simulink model "DCHR_Dispatch_Stateflow_v22"  (R2026a)
settings: Solver=FixedStepDiscrete  StopTime=dchr_stop_v22  FixedStep=dchr_dt_v22
model workspace (MAT data in the model file):
  dchr_E0_v22 = 0
  dchr_dt_v22 = 1
  dchr_h_v22 = [8 0.45 1.2 8 0.08 0 4 0 0]
  dchr_input_v22 = [0  6  35  70  5; 1  0  35  70  6; 2  0  35  70  10]
  dchr_p_v22 = [1 10 3 4 0.9 0.8 0.01 2]
  dchr_stop_v22 = 2
settings Model: Creator=Lysda  LastModifiedBy=Lysda

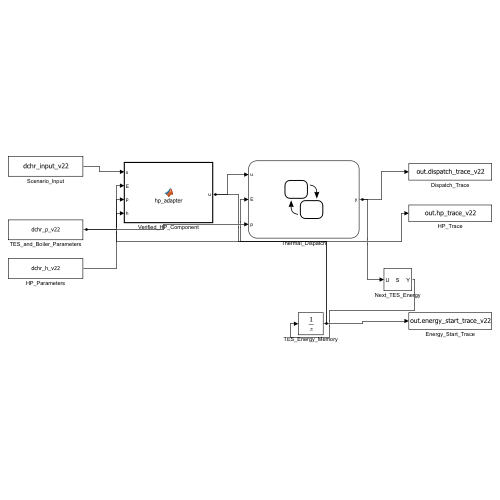
[thumbnail: Simulink's stored preview of the top-level diagram]
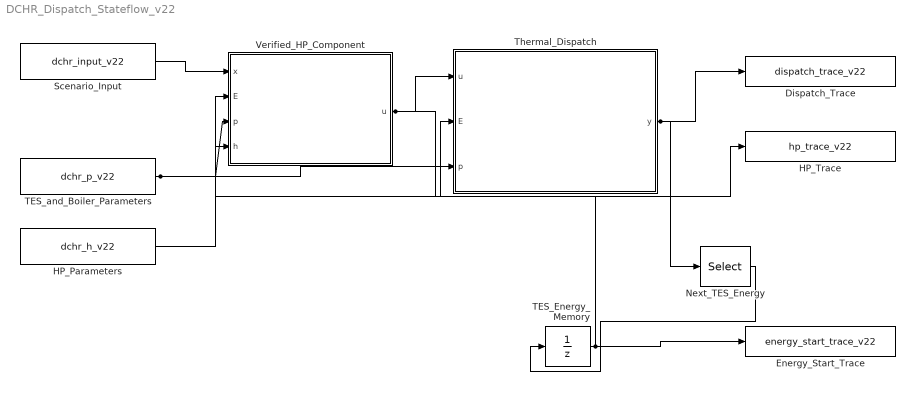
== system DCHR_Dispatch_Stateflow_v22 ==
  Dispatch_Trace : ToWorkspace  VariableName=dispatch_trace_v22  SaveFormat=Timeseries  SampleTime=-1
  Energy_Start_Trace : ToWorkspace  VariableName=energy_start_trace_v22  SaveFormat=Timeseries  SampleTime=-1
  HP_Parameters : Constant  Value=dchr_h_v22
  HP_Trace : ToWorkspace  VariableName=hp_trace_v22  SaveFormat=Timeseries  SampleTime=-1
  Next_TES_Energy : Selector  InputPortWidth=13  IndexOptions=Index vector (dialog)  Indices=8  OutputSizes=1
  Scenario_Input : FromWorkspace  VariableName=dchr_input_v22  SampleTime=dchr_dt_v22  Interpolate=off  OutputAfterFinalValue=Holding final value
  TES_Energy_Memory : UnitDelay  InitialCondition=dchr_E0_v22  SampleTime=dchr_dt_v22
  TES_and_Boiler_Parameters : Constant  Value=dchr_p_v22
  Thermal_Dispatch : Stateflow chart  TreatAsAtomicUnit=on
  Verified_HP_Component : MATLAB Function  TreatAsAtomicUnit=on
  wires:
  Scenario_Input/1 -> Verified_HP_Component/1(x)
  TES_Energy_Memory/1 -> Verified_HP_Component/2(E), Thermal_Dispatch/2(E), Energy_Start_Trace/1
  TES_and_Boiler_Parameters/1 -> Verified_HP_Component/3(p), Thermal_Dispatch/3(p)
  HP_Parameters/1 -> Verified_HP_Component/4(h)
  Verified_HP_Component/1(u) -> Thermal_Dispatch/1(u), HP_Trace/1
  Thermal_Dispatch/1(y) -> Next_TES_Energy/1, Dispatch_Trace/1
  Next_TES_Energy/1 -> TES_Energy_Memory/1

== matlab function DCHR_Dispatch_Stateflow_v22/Verified_HP_Component ==
  data: x input; u output; E input; p input; h input
function u=hp_adapter(x,E,p,h)
%#codegen
coder.extrinsic('dchr_stateflow_hp_v22');
u=zeros(8,1);
u=dchr_stateflow_hp_v22(x,E,p,h);
end

== stateflow chart DCHR_Dispatch_Stateflow_v22/Thermal_Dispatch ==
  settings: updateMethod=DISCRETE  sampleTime=dchr_dt_v22  description=v22 six-state finite TES/HP/boiler dispatch. Normal-mode host HP component; state actions drive all delivery ports.
  state IDLE
    en,du:
    y=stateflow_allocate_v22(0,u,E,p);
  state HEAT_RECOVERY
    en,du:
    y=stateflow_allocate_v22(1,u,E,p);
  state STORAGE_CHARGE
    en,du:
    y=stateflow_allocate_v22(2,u,E,p);
  state STORAGE_DISCHARGE
    en,du:
    y=stateflow_allocate_v22(3,u,E,p);
  state BACKUP
    en,du:
    y=stateflow_allocate_v22(4,u,E,p);
  state UNMET_DEMAND
    en,du:
    y=stateflow_allocate_v22(5,u,E,p);
  (junction 22) -> STORAGE_CHARGE [order 3] : [stateflow_choose_mode_v22(u,E,p)==2]
  (junction 22) -> HEAT_RECOVERY [order 2] : [stateflow_choose_mode_v22(u,E,p)==1]
  (default) -> (junction 22)
  (junction 22) -> IDLE [order 1] : [stateflow_choose_mode_v22(u,E,p)==0]
  (junction 22) -> UNMET_DEMAND [order 6] : [stateflow_choose_mode_v22(u,E,p)==5]
  (junction 22) -> STORAGE_DISCHARGE [order 4] : [stateflow_choose_mode_v22(u,E,p)==3]
  (junction 22) -> BACKUP [order 5] : [stateflow_choose_mode_v22(u,E,p)==4]
  STORAGE_CHARGE -> STORAGE_DISCHARGE [order 3] : [stateflow_choose_mode_v22(u,E,p)==3]
  HEAT_RECOVERY -> STORAGE_DISCHARGE [order 3] : [stateflow_choose_mode_v22(u,E,p)==3]
  STORAGE_CHARGE -> BACKUP [order 4] : [stateflow_choose_mode_v22(u,E,p)==4]
  STORAGE_DISCHARGE -> IDLE [order 1] : [stateflow_choose_mode_v22(u,E,p)==0]
  UNMET_DEMAND -> IDLE [order 1] : [stateflow_choose_mode_v22(u,E,p)==0]
  STORAGE_CHARGE -> IDLE [order 1] : [stateflow_choose_mode_v22(u,E,p)==0]
  BACKUP -> IDLE [order 1] : [stateflow_choose_mode_v22(u,E,p)==0]
  HEAT_RECOVERY -> IDLE [order 1] : [stateflow_choose_mode_v22(u,E,p)==0]
  STORAGE_DISCHARGE -> HEAT_RECOVERY [order 2] : [stateflow_choose_mode_v22(u,E,p)==1]
  STORAGE_DISCHARGE -> STORAGE_CHARGE [order 3] : [stateflow_choose_mode_v22(u,E,p)==2]
  BACKUP -> HEAT_RECOVERY [order 2] : [stateflow_choose_mode_v22(u,E,p)==1]
  IDLE -> HEAT_RECOVERY [order 1] : [stateflow_choose_mode_v22(u,E,p)==1]
  IDLE -> STORAGE_CHARGE [order 2] : [stateflow_choose_mode_v22(u,E,p)==2]
  UNMET_DEMAND -> HEAT_RECOVERY [order 2] : [stateflow_choose_mode_v22(u,E,p)==1]
  STORAGE_CHARGE -> HEAT_RECOVERY [order 2] : [stateflow_choose_mode_v22(u,E,p)==1]
  BACKUP -> STORAGE_CHARGE [order 3] : [stateflow_choose_mode_v22(u,E,p)==2]
  UNMET_DEMAND -> STORAGE_CHARGE [order 3] : [stateflow_choose_mode_v22(u,E,p)==2]
  HEAT_RECOVERY -> STORAGE_CHARGE [order 2] : [stateflow_choose_mode_v22(u,E,p)==2]
  IDLE -> STORAGE_DISCHARGE [order 3] : [stateflow_choose_mode_v22(u,E,p)==3]
  HEAT_RECOVERY -> BACKUP [order 4] : [stateflow_choose_mode_v22(u,E,p)==4]
  STORAGE_CHARGE -> UNMET_DEMAND [order 5] : [stateflow_choose_mode_v22(u,E,p)==5]
  IDLE -> BACKUP [order 4] : [stateflow_choose_mode_v22(u,E,p)==4]
  IDLE -> UNMET_DEMAND [order 5] : [stateflow_choose_mode_v22(u,E,p)==5]
  HEAT_RECOVERY -> UNMET_DEMAND [order 5] : [stateflow_choose_mode_v22(u,E,p)==5]
  UNMET_DEMAND -> STORAGE_DISCHARGE [order 4] : [stateflow_choose_mode_v22(u,E,p)==3]
  BACKUP -> STORAGE_DISCHARGE [order 4] : [stateflow_choose_mode_v22(u,E,p)==3]
  STORAGE_DISCHARGE -> BACKUP [order 4] : [stateflow_choose_mode_v22(u,E,p)==4]
  STORAGE_DISCHARGE -> UNMET_DEMAND [order 5] : [stateflow_choose_mode_v22(u,E,p)==5]
  UNMET_DEMAND -> BACKUP [order 5] : [stateflow_choose_mode_v22(u,E,p)==4]
  BACKUP -> UNMET_DEMAND [order 5] : [stateflow_choose_mode_v22(u,E,p)==5]
  data: u function_input; E function_input; p function_input; mode function_output; mode function_input; u function_input; E function_input; p function_input; y function_output; u input double size=[8 1]; E input double size=1; p input double size=[1 8]; y output double size=[13 1]
  function mode = stateflow_choose_mode_v22(u,E,p):
    | function mode = stateflow_choose_mode_v22(u,E,p)
    | %#codegen
    | % Highest service condition; BACKUP/UNMET can include HP and TES discharge.
    | % u = [demand, HP heat, electricity, source used, request, COP, available, unused]
    | % p = [dt_h, capacity, charge limit, discharge limit, etaC, etaD, loss/h, boiler]
    | after=E*(1-p(7)*p(1));
    | direct=min(u(1),u(2));
    | discharge=min([max(0,u(1)-direct),p(4),after*p(6)/p(1)]);
    | remaining=max(0,u(1)-direct-discharge);
    | if remaining>p(8)
    |     mode=5;
    | elseif remaining>0
    |     mode=4;
    | elseif discharge>0
    |     mode=3;
    | elseif u(2)>direct
    |     mode=2;
    | elseif direct>0
    |     mode=1;
    | else
    |     mode=0;
    | end
    | end
  function y = stateflow_allocate_v22(mode,u,E,p):
    | function y = stateflow_allocate_v22(mode,u,E,p)
    | %#codegen
    | % Called by the active Stateflow state's entry and during actions.
    | % States determine which TES/backup/unmet ports may operate.
    | dt=p(1); after=E*(1-p(7)*dt);
    | direct=0; charge=0; discharge=0; gas=0; unmet=0;
    | if mode>=1
    |     direct=min(u(1),u(2));
    | end
    | if mode==2
    |     charge=min([max(0,u(2)-direct),p(3),(p(2)-after)/dt/p(5)]);
    | end
    | if mode>=3
    |     discharge=min([max(0,u(1)-direct),p(4),after*p(6)/dt]);
    | end
    | if mode>=4
    |     gas=min(p(8),max(0,u(1)-direct-discharge));
    | end
    | if mode==5
    |     unmet=max(0,u(1)-direct-discharge-gas);
    | end
    | next=min(p(2),max(0,after+p(5)*charge*dt-discharge*dt/p(6)));
    | standing=E-after;
    | chargeLoss=(1-p(5))*charge*dt;
    | dischargeLoss=discharge*dt/p(6)-discharge*dt;
    | supplied=direct+discharge+gas;
    | residual=(u(4)+u(3)+gas)*dt+E-supplied*dt-next-standing-chargeLoss-dischargeLoss;
    | y=[mode;direct;charge;discharge;gas;unmet;after;next;standing;chargeLoss;dischargeLoss;supplied;residual];
    | end
